simulink model "pid_board_bench"  (R2024b)
settings: Solver=ode4  StartTime=0.0  StopTime=pbsim.t_stop  FixedStep=pcb.sim_dt  RelTol=1e-3
PostLoadFcn:
  | pbdir_ = fileparts(get_param('pid_board_bench', 'FileName')); if ~exist('pcb', 'var'), run(fullfile(pbdir_, 'pid_board_params.m')); end; if ~exist('CtrlIn', 'var'), run(fullfile(pbdir_, '..', 'common', 'quad_ctrl_buses.m')); end; clear pbdir_
Description:
  | Bench harness: pbsim.bench_in from pid_board_bench_inputs. Test points (U_ROLL, roll_E, roll_I, PLANT_OUT_ROLL, ...) are in logsout / Simulation Data Inspector.
settings Model: Creator=doubi  LastModifiedBy=doubi

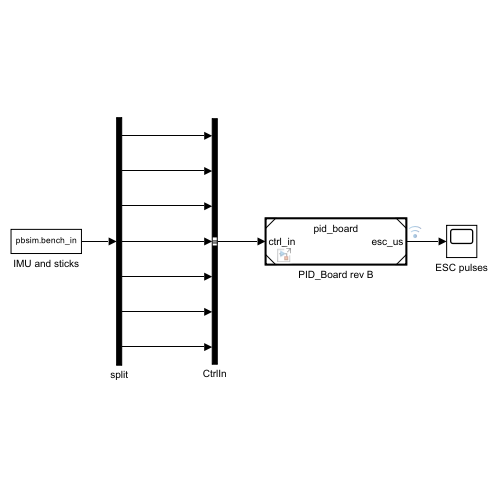
[thumbnail: Simulink's stored preview of the top-level diagram]
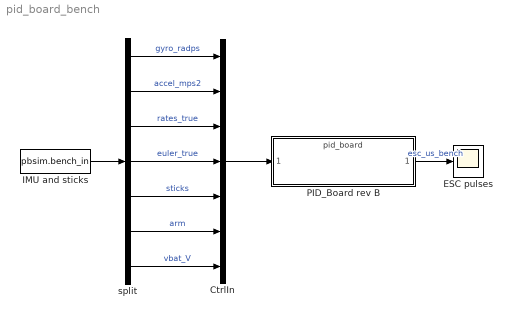
== system pid_board_bench ==
  CtrlIn : BusCreator  Inputs=7  OutDataTypeStr=Bus: CtrlIn
      settings: InheritFromInputs=off
  ESC pulses : Scope
  IMU and sticks : FromWorkspace  VariableName=pbsim.bench_in  SampleTime=1e-3  OutputAfterFinalValue=Holding final value
  PID_Board rev B : ModelReference  ModelNameDialog=pid_board  ParameterArgumentNames=board_variant  ParameterArgumentValues=pcb.variant  UsingDefaultArgumentValue=0  SimulationMode=Normal  ModelReferenceVersion=1.1
  split : Demux  Outputs=[3 3 3 3 4 1 1]
  wires:
  split/6 -> CtrlIn/6  "arm"
  split/4 -> CtrlIn/4  "euler_true"
  split/2 -> CtrlIn/2  "accel_mps2"
  IMU and sticks/1 -> split/1
  split/7 -> CtrlIn/7  "vbat_V"
  split/5 -> CtrlIn/5  "sticks"
  split/3 -> CtrlIn/3  "rates_true"
  split/1 -> CtrlIn/1  "gyro_radps"
  CtrlIn/1 -> PID_Board rev B/1
  PID_Board rev B/1 -> ESC pulses/1  "esc_us_bench"
